simulink model "normal"  (R2026b)
settings: Solver=ode23s  StopTime=T_sim  MaxStep=1e-3  MinStep=1e-6  RelTol=1e-5
InitFcn:
  | run param_file_2.m
values from neighbouring files (symbols this model uses):
  param = struct()    [param_file.m]    (also in param_file_2.m)
settings Model: Creator=user  LastModifiedBy=mahmu
settings SolverCC: ZeroCrossAlgorithm=Adaptive
settings DebuggingCC: IgnoredZcDiagnostic=none
settings RTWCC: GPUComputeCapability=5.0
settings SimscapeCC: SimscapeUseEnergyAccounting=off

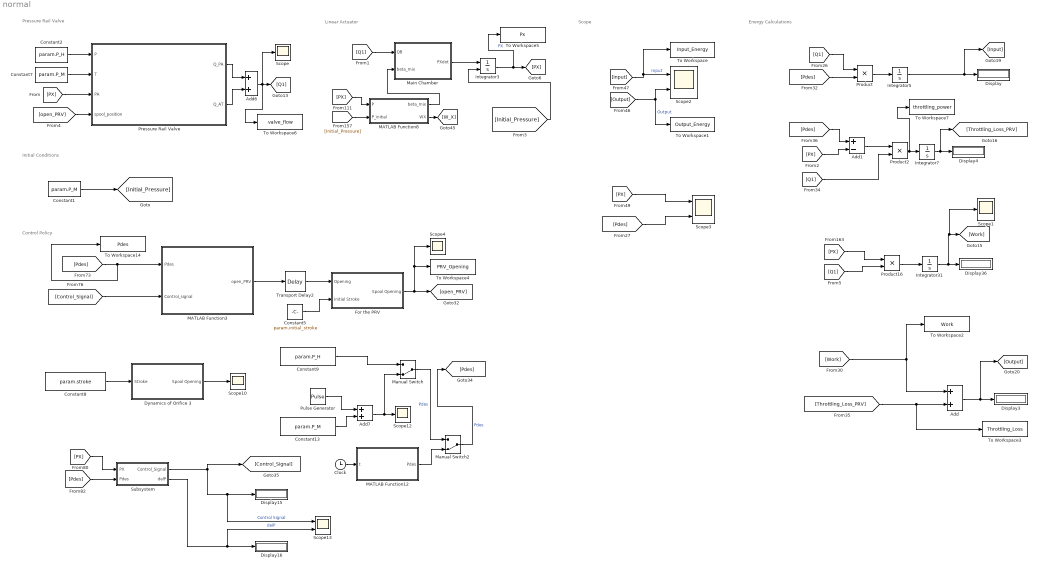
== system normal ==
  note: Control Policy
  note: Energy Calculations
  note: Pressure Rail Valve
  note: Scope
  note: Initial Conditions
  note: Linear Actuator
  Add : Sum
  Add1 : Sum  Inputs=+-
  Add6 : Sum
  Add7 : Sum
  Clock : Clock
  Constant1 : Constant  Value=param.P_M
  Constant13 : Constant  Value=param.P_M
  Constant2 : Constant  Value=param.P_H
  Constant5 : Constant  Value=param.initial_stroke
  Constant7 : Constant  Value=param.P_M
  Constant8 : Constant  Value=param.stroke
  Constant9 : Constant  Value=param.P_H
  Display{,3..4,15..16,36} (6 alike) : Display
  Dynamics of Orifice 3 : Subsystem
  For the PRV : Subsystem
  Integrator3 : Integrator  InitialConditionSource=external
  Integrator31 : Integrator
  Integrator5 : Integrator
  Integrator7 : Integrator
  MATLAB Function12 : MATLAB Function  TreatAsAtomicUnit=on
  MATLAB Function3 : MATLAB Function  TreatAsAtomicUnit=on
  MATLAB Function8 : MATLAB Function  TreatAsAtomicUnit=on
  Main Chamber : MATLAB Function  TreatAsAtomicUnit=on
  Manual Switch : ManualSwitch  CurrentSetting=0
  Manual Switch2 : ManualSwitch  CurrentSetting=0
  Pressure Rail Valve : MATLAB Function  TreatAsAtomicUnit=on
  Product : Product
  Product16 : Product
  Product2 : Product
  Pulse Generator : DiscretePulseGenerator  PulseType=Time based  Amplitude=param.P_H-param.P_M  Period=param.T_period  PulseWidth=50  PhaseDelay=param.delay
  Scope{,1,4,10,12} (5 alike) : Scope
      Scope settings: ActiveDisplayYMinimum=-3.0902796801951923E-5  ActiveDisplayYMaximum=0.00027812517121756736  DataLoggingVariableName=ScopeData14
      Scope1 settings: ActiveDisplayYMinimum=-0.970213268051517  ActiveDisplayYMaximum=8.7319194124636539
      Scope10 settings: ActiveDisplayYMinimum=-0.00062  ActiveDisplayYMaximum=0.00562  DataLoggingVariableName=ScopeData9
      Scope12 settings: ActiveDisplayYMinimum=2.585125E+6  ActiveDisplayYMaximum=1.1203875E+7  DataLoggingVariableName=ScopeData11
      Scope4 settings: ActiveDisplayYMinimum=-0.12499999999998967  ActiveDisplayYMaximum=1.1249999999999074  DataLoggingVariableName=ScopeData3
  Scope13 : Scope  NumInputPorts=2
      settings: ActiveDisplayYMinimum=-0.12499999999999997  ActiveDisplayYMaximum=1.125  DataLoggingVariableName=ScopeData12
  Scope2 : Scope  NumInputPorts=2
      settings: ActiveDisplayYMinimum=-1.5404482275164069  ActiveDisplayYMaximum=13.864034047647666
  Scope3 : Scope  NumInputPorts=2
      settings: ActiveDisplayYMinimum=-38180.936985161854  ActiveDisplayYMaximum=1.3423951077997142E+7  DataLoggingVariableName=ScopeData2
  Subsystem : Subsystem
  To Workspace : ToWorkspace  VariableName=Input_Energy  SaveFormat=Timeseries  SampleTime=-1
  To Workspace1 : ToWorkspace  VariableName=Output_Energy  SaveFormat=Timeseries  SampleTime=-1
  To Workspace14 : ToWorkspace  VariableName=Pdes  SaveFormat=Timeseries  SampleTime=-1
  To Workspace2 : ToWorkspace  VariableName=Work  SaveFormat=Timeseries  SampleTime=-1
  To Workspace3 : ToWorkspace  VariableName=Throttling_Loss  SaveFormat=Timeseries  SampleTime=-1
  To Workspace4 : ToWorkspace  VariableName=PRV_Opening  SaveFormat=Timeseries  SampleTime=-1
  To Workspace5 : ToWorkspace  VariableName=Px  SaveFormat=Timeseries  SampleTime=-1
  To Workspace6 : ToWorkspace  VariableName=valve_flow  SaveFormat=Timeseries  SampleTime=-1
  To Workspace7 : ToWorkspace  VariableName=throttling_power  SaveFormat=Timeseries  SampleTime=-1
  Transport Delay2 : TransportDelay  DelayTime=param.delay_switch  InitialOutput=param.initial_stroke  BufferSize=1024*105
  wires:
  Constant2/1 -> Pressure Rail Valve/1(P)
  Constant1/1 -> [Initial_Pressure]
  Main Chamber/1(PXdot) -> Integrator3/1
  [Initial_Pressure] -> Integrator3/2
  Integrator3/1 -> To Workspace5/1, [PX]  "PX"
  [Q1] -> Main Chamber/1(QB)
  [Q1] -> Product/1
  [Pdes] -> Product/2
  Product/1 -> Integrator5/1
  [Work] -> To Workspace2/1, Add/1
  Add/1 -> [Output], Display3/1
  [PX] -> Add1/2
  Add1/1 -> Product2/1
  [Q1] -> Product2/2
  Product2/1 -> To Workspace7/1, Integrator7/1
  Integrator7/1 -> [Throttling_Loss_PRV], Display4/1
  [Input] -> Scope2/1, To Workspace/1  "Input"
  [Output] -> To Workspace1/1, Scope2/2  "Output"
  [Throttling_Loss_PRV] -> To Workspace3/1, Add/2
  [PX] -> Scope3/1
  [Pdes] -> Scope3/2
  For the PRV/1(Spool Opening) -> To Workspace4/1, Scope4/1, [open_PRV]
  [Control_Signal] -> MATLAB Function3/2(Control_signal)
  Transport Delay2/1 -> For the PRV/1(Opening)
  MATLAB Function3/1(open_PRV) -> Transport Delay2/1
  Pressure Rail Valve/1(Q_PA) -> Add6/1
  Pressure Rail Valve/2(Q_AT) -> Add6/2
  Add6/1 -> To Workspace6/1, [Q1], Scope/1
  [PX] -> Pressure Rail Valve/3(PA)
  Constant7/1 -> Pressure Rail Valve/2(T)
  [open_PRV] -> Pressure Rail Valve/4(spool_position)
  [Pdes] -> Subsystem/2(Pdes)
  [PX] -> Subsystem/1(PX)
  Subsystem/1(Control_Signal) -> Scope13/1, Display15/1, [Control_Signal]  "Control Signal"
  Subsystem/2(delP) -> Scope13/2, Display16/1  "delP"
  Constant9/1 -> Manual Switch/1
  Constant13/1 -> Add7/2
  Pulse Generator/1 -> Add7/1
  Add7/1 -> Manual Switch/2, Scope12/1
  Dynamics of Orifice 3/1(Spool Opening) -> Scope10/1
  Constant8/1 -> Dynamics of Orifice 3/1(Stroke)
  [Pdes] -> To Workspace14/1, MATLAB Function3/1(Pdes)
  [Pdes] -> Add1/1
  Integrator5/1 -> [Input], Display/1
  Constant5/1 -> For the PRV/2(Initial Stroke)
  MATLAB Function8/1(beta_mix) -> Main Chamber/2(beta_mix)
  [PX] -> MATLAB Function8/1(P)
  MATLAB Function8/2(WX) -> [W_X]
  [Initial_Pressure] -> MATLAB Function8/2(P_initial)
  [Q1] -> Product16/2
  [PX] -> Product16/1
  Product16/1 -> Integrator31/1
  Integrator31/1 -> Scope1/1, [Work], Display36/1
  MATLAB Function12/1(Pdes) -> Manual Switch2/2
  Manual Switch/1 -> Manual Switch2/1  "Pdes"
  Manual Switch2/1 -> [Pdes]  "Pdes"
  Clock/1 -> MATLAB Function12/1(t)

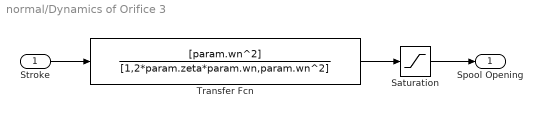
== system normal/Dynamics of Orifice 3 ==
  Stroke : Inport
  Saturation : Saturate  UpperLimit=param.stroke  LowerLimit=0
  Transfer Fcn : TransferFcn  Numerator=[param.wn^2]  Denominator=[1,2*param.zeta*param.wn,param.wn^2]
  Spool Opening : Outport
  wires:
  Transfer Fcn/1 -> Saturation/1
  Saturation/1 -> Spool Opening/1
  Stroke/1 -> Transfer Fcn/1

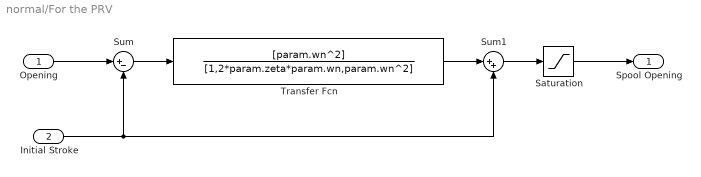
== system normal/For the PRV ==
  Opening : Inport
  Initial Stroke : Inport  Port=2
  Saturation : Saturate  UpperLimit=1  LowerLimit=-1
  Sum : Sum  Inputs=|+-
  Sum1 : Sum  Inputs=|++
  Transfer Fcn : TransferFcn  Numerator=[param.wn^2]  Denominator=[1,2*param.zeta*param.wn,param.wn^2]
  Spool Opening : Outport
  wires:
  Saturation/1 -> Spool Opening/1
  Sum1/1 -> Saturation/1
  Transfer Fcn/1 -> Sum1/1
  Sum/1 -> Transfer Fcn/1
  Opening/1 -> Sum/1
  Initial Stroke/1 -> Sum1/2, Sum/2

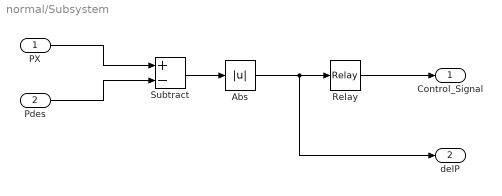
== system normal/Subsystem ==
  PX : Inport
  Pdes : Inport  Port=2
  Abs : Abs  SaturateOnIntegerOverflow=off
  Relay : Relay  OnSwitchValue=15e5  OffSwitchValue=1e4  OnOutputValue=0  OffOutputValue=1
  Subtract : Sum  Inputs=+-
  Control_Signal : Outport
  delP : Outport  Port=2
  wires:
  PX/1 -> Subtract/1
  Pdes/1 -> Subtract/2
  Subtract/1 -> Abs/1
  Abs/1 -> delP/1, Relay/1
  Relay/1 -> Control_Signal/1

== matlab function normal/Pressure Rail Valve ==
  data: P input; T input; Q_PA output; Q_AT output; PA input; spool_position input; param parameter
function [Q_PA, Q_AT] = RailValve(P, T, PA, spool_position, param)

db = param.valve_buffer;

spool_position = max(-1, min(1, spool_position));

if abs(spool_position) <= db
    f = 0;
else
    f = (abs(spool_position) - db) / (1 - db);
    f = max(0, min(1, f));
end

A_PA = 0;
A_AT = 0;

if spool_position > db
    A_PA = param.max_Avt * f;
elseif spool_position < -db
    A_AT = param.max_Avt * f;
end

Q_PA = param.Cd * A_PA * sqrt(2/param.rho) * sqrt(abs(P-PA)) * sign(P-PA);
Q_AT = param.Cd * A_AT * sqrt(2/param.rho) * sqrt(abs(PA-T)) * sign(T-PA);

end

== matlab function normal/Main Chamber ==
  data: QB input; PXdot output; param parameter; beta_mix input
function PXdot = Main_Chamber(QB, param, beta_mix)

Vx = param.VA_0 + param.VT_0 + param.VP_0 + param.V1_0;
PXdot = (beta_mix/Vx)*(QB);

== matlab function normal/MATLAB Function3 ==
  data: Pdes input; open_PRV output; param parameter; Control_signal input
function open_PRV  = fcn(Pdes, param, Control_signal)

if Pdes == param.P_H && Control_signal == 0
    open_PRV = 1;
elseif Pdes == param.P_M && Control_signal == 0
    open_PRV = -1;
elseif Pdes == param.P_H && Control_signal > 0
    open_PRV = 1;
elseif Pdes == param.P_M && Control_signal > 0
    open_PRV = -1;
else
    open_PRV = 0;
end

== matlab function normal/MATLAB Function8 ==
  data: P input; P_initial input; beta_mix output; param parameter; WX output
function [beta_mix, WX] = oil_comp(P,P_initial,param)

%Ph=7e6, P0=1e5
Pg = P-param.P_T;   % Gauge pressure
r = P/param.P_T;    % Pressure ratio
e = exp(Pg/param.beta); 
rv = (1./e+param.air*r.^(-1/param.gamma))/(1+param.air);      %Volume ratio

beta_mix = rv*(1+param.air)/(1/(e*param.beta)+...
           param.air/(param.gamma*param.P_T*r^(1/param.gamma+1)));

El = param.beta*(e - (1 + Pg/param.beta)) + param.P_T*(e - 1);              % Energy in liquid
Eg = P/(param.gamma - 1) .* (1 - r.^(1/param.gamma - 1));           % Energy in gas
E  = (El./e + param.air*Eg.*r.^(-1/param.gamma)) ./ ...
     (1./e + param.air*r.^(-1/param.gamma));                       % Energy in mixture
WX  = E - (1./rv - 1)*P_initial;                                 % Compressibility energy density

== matlab function normal/MATLAB Function12 ==
  data: t input; Pdes output; param parameter
function Pdes = fcn(t, param)

% t = clock_time(1);
% 
% if (t >= 0.20 && t < 0.75) || ...
%         (t >= 1.30 && t < 1.85) || ...
%         t >= 2.40
%     Pdes = param.P_H;
% else
%     Pdes = param.P_M;
% end
% 
% end
% t = clock_time(1);

if t < 0.20
    Pdes = param.P_M;
elseif t < 0.75
    Pdes = param.P_H;
elseif t < 1.30
    Pdes = param.P_M;
else
    Pdes = param.P_H;
end

end

% function Pdes = fcn(clock_time, param)
% 
% if (clock_time >= 0.20 && clock_time < 0.75) || ...
%         (clock_time >= 1.30 && clock_time < 1.85)
%     Pdes = param.P_H;
% else
%     Pdes = param.P_M;
% end
% 
% end
